simulink model "MPPT_p0x26oPartIALShadingFD"  (R2024b)
settings: Solver=VariableStepAuto  StartTime=0.0  StopTime=1  FixedStep=1e-6  RelTol=1e-4
libraries: spsDiodeLib x5, spsPVArrayLib x4, spsSeriesRLCBranchLib x4, spsVoltageMeasurementLib x3, spsCurrentMeasurementLib x2, spsMosfetLib x1, simulink x1, sps_lib x1
settings Model: Creator=VICTUS  LastModifiedBy=VICTUS
settings SolverCC: ZeroCrossAlgorithm=Adaptive
settings DebuggingCC: MaskedZcDiagnostic=none  IgnoredZcDiagnostic=none

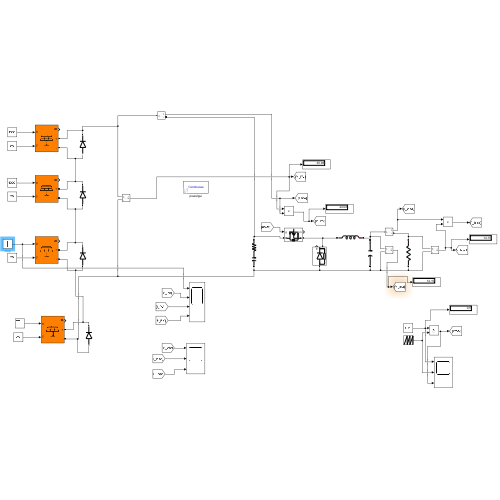
[thumbnail: Simulink's stored preview of the top-level diagram]
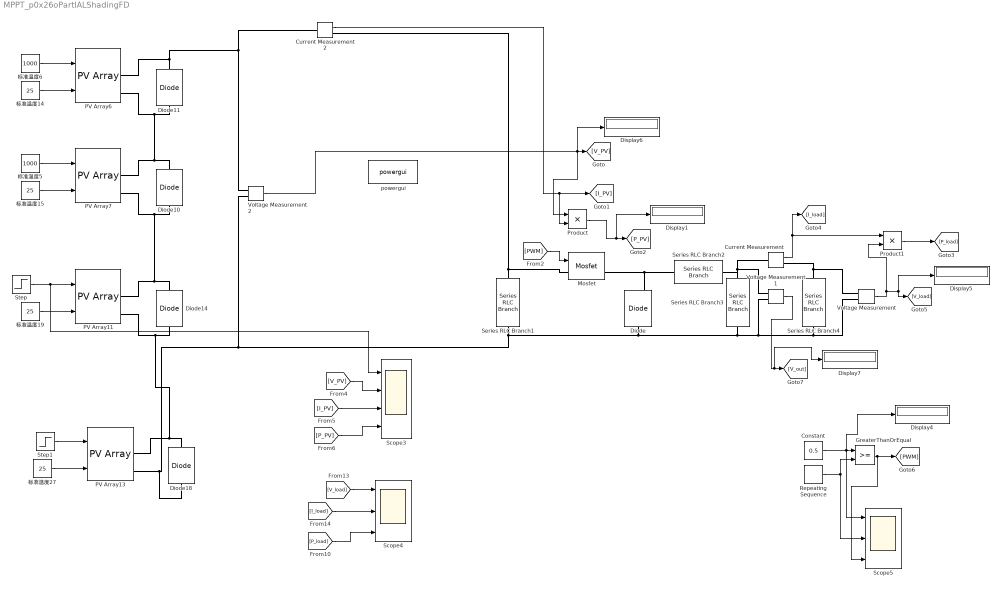
== system MPPT_p0x26oPartIALShadingFD ==
  Constant : Constant  Value=0.5
  Current Measurement : spsCurrentMeasurementLib/Current Measurement  PhasorSimulation=off  OutputType=Complex  PSBequivalent=0
  Current Measurement2 : spsCurrentMeasurementLib/Current Measurement  PhasorSimulation=off  OutputType=Complex  PSBequivalent=0
  Diode : spsDiodeLib/Diode  Ron=0.001  Lon=0  Vf=0.8  IC=0  UseSnubber=0  Rs=500  Cs=250e-9  Measurements=on
  Diode{10..11,14,18} (4 alike) : spsDiodeLib/Diode  Ron=0.001  Lon=0  Vf=0.8  IC=0  UseSnubber=off  Rs=inf  Cs=250e-9  Measurements=off
  Display{1,4..7} (5 alike) : Display
  GreaterThanOrEqual : RelationalOperator  OutDataTypeStr=boolean  RndMeth=Simplest  InputSameDT=off
  Mosfet : spsMosfetLib/Mosfet  Ron=0.1  Lon=0  Rd=0.01  Vfd=0  IC=0  Rs=1e5  Cs=inf  Measurements=on
  PV Array{6..7,11,13} (4 alike) : spsPVArrayLib/PV Array  Npar=1  Nser=1  PlotType=array @ 1000 W/m2 & specified temperatures  S_vec="[ 1000  500  100 ]"  Temp_C_vec="[ 45 25  ]"  ModuleName=User-defined  PlotWhenSelected=off  Pm=120.75  Ncell=16  Voc=22  Isc=7.5  Vm=17.5  Im=6.9  beta_Voc_pc=-0.36099  alpha_Isc_pc=0.102  beta_Voc=-0.079418  alpha_Isc=0.00765  IL=7.6829  I0=2.1898e-10  nI=2.2089  Rsh=50.0358  Rs=0.26399  RobustModel=off  RobustCellTemperature=313.3991  BAL=off  Tc=1e-6  Tfilter=5e-5
  Product : Product
  Product1 : Product
  Repeating Sequence : simulink/Sources/Repeating Sequence  rep_seq_t=[0 2e-4]  rep_seq_y=[0 1]
  Scope3 : Scope  NumInputPorts=4
  Scope4 : Scope  NumInputPorts=3
  Scope5 : Scope  NumInputPorts=3
  Series RLC Branch1 : spsSeriesRLCBranchLib/Series RLC Branch  LConnTagsString=__new0  RConnTagsString=__new0  BranchType=RC  Resistance=0.001  Inductance=1e-3  SetiL0=off  InitialCurrent=0  Capacitance=338e-6  Setx0=off  InitialVoltage=0  Measurements=None
  Series RLC Branch2 : spsSeriesRLCBranchLib/Series RLC Branch  LConnTagsString=__new0  RConnTagsString=__new0  BranchType=L  Resistance=0.001  Inductance=1.25e-3  SetiL0=off  InitialCurrent=0  Capacitance=1000e-6  Setx0=off  InitialVoltage=0  Measurements=None
  Series RLC Branch3 : spsSeriesRLCBranchLib/Series RLC Branch  LConnTagsString=__new0  RConnTagsString=__new0  BranchType=C  Resistance=0.001  Inductance=1e-3  SetiL0=off  InitialCurrent=0  Capacitance=187.5e-6  Setx0=off  InitialVoltage=0  Measurements=None
  Series RLC Branch4 : spsSeriesRLCBranchLib/Series RLC Branch  LConnTagsString=__new0  RConnTagsString=__new0  BranchType=R  Resistance=1  Inductance=1e-3  SetiL0=off  InitialCurrent=0  Capacitance=1000e-6  Setx0=off  InitialVoltage=0  Measurements=None
  Step : Step  Time=0.5  Before=1000  After=400  SampleTime=0
  Step1 : Step  Time=0.5  Before=1000  After=400  SampleTime=0
  Voltage Measurement : spsVoltageMeasurementLib/Voltage Measurement  PhasorSimulation=off  OutputType=Complex  PSBequivalent=0
  Voltage Measurement1 : spsVoltageMeasurementLib/Voltage Measurement  PhasorSimulation=off  OutputType=Complex  PSBequivalent=0
  Voltage Measurement2 : spsVoltageMeasurementLib/Voltage Measurement  PhasorSimulation=off  OutputType=Complex  PSBequivalent=0
  powergui : sps_lib/powergui  Priority=1  SimulationMode=Continuous  SampleTime=50e-6  frequency=60  Iterations=50  frequencyindice=0  Pbase=100e6  ErrMax=1e-4  UnitsV=kV  UnitsW=MW  buscounter=0  FunctionMessages=off  echomessages=off  EnableUseOfTLC=off  CurrentSourceSwitches=off  DisableSnubberDevices=off  DisableRonSwitches=off  DisableVfSwitches=off  DisplayEquations=off  AutomaticDiscreteSolvers=off  SolverType=Tustin/Backward Euler (TBE)  Interpol=off  ExternalGateDelay=off  methode=off  Ts=100  x0status=blocks  SPID=on  SwTol=0  HookPort=off  NonlinearTolerance=1e-4  nMaxIteration=100  ContinueOnMaxIteration=off  RestoreLinks=warning  ResistiveCurrentMeasurement=off  Frange=[0:2:500]  Ylog=off  Xlog=on  ShowGrid=off  save=off  variable=ZData  structure=0  ZoomFFT=off  StartTime=0.0  cycles=1  DisplayStyle=1  fundamental=60  FreqAxis=off  MaxFrequency=1000  frequencyindicesteady=1  RmsSteady=1  display=off
  标准温度{14..15,19,27} (4 alike) : Constant  Value=25  SampleTime=0.001
  标准温度5 : Constant  Value=1000  SampleTime=0.001
  标准温度6 : Constant  Value=1000  SampleTime=0.001
  wires:
  标准温度5/1 -> PV Array7/1
  [V_load] -> Scope4/1
  [PWM] -> Mosfet/1
  Product1/1 -> [P_load]
  [I_PV] -> Scope3/3
  Voltage Measurement2/1 -> Product/1, Display6/1, [V_PV]
  标准温度14/1 -> PV Array6/2
  Voltage Measurement/1 -> Product1/2, Display5/1, [V_load]
  [I_load] -> Scope4/2
  标准温度27/1 -> PV Array13/2
  Current Measurement/1 -> [I_load], Product1/1
  Current Measurement2/1 -> Product/2, [I_PV]
  标准温度15/1 -> PV Array7/2
  标准温度6/1 -> PV Array6/1
  [P_load] -> Scope4/3
  Step/1 -> Scope3/1, PV Array11/1
  Product/1 -> Display1/1, [P_PV]
  标准温度19/1 -> PV Array11/2
  [V_PV] -> Scope3/2
  Voltage Measurement1/1 -> Display7/1, [V_out]
  [P_PV] -> Scope3/4
  Step1/1 -> PV Array13/1
  GreaterThanOrEqual/1 -> Scope5/3, [PWM]
  Repeating Sequence/1 -> Scope5/2, GreaterThanOrEqual/2
  Constant/1 -> Scope5/1, GreaterThanOrEqual/1, Display4/1
  connections:
  Voltage Measurement2/LConn1 -- PV Array6/RConn1 -- Diode11/RConn1 -- Current Measurement2/LConn1
  Voltage Measurement/LConn1 -- Series RLC Branch4/LConn1 -- Current Measurement/RConn1
  PV Array7/RConn2 -- Diode14/RConn1 -- PV Array11/RConn1 -- Diode10/LConn1
  Series RLC Branch2/RConn1 -- Diode/RConn1 -- Mosfet/RConn1
  Series RLC Branch3/LConn1 -- Current Measurement/LConn1 -- Series RLC Branch2/LConn1 -- Voltage Measurement1/LConn1
  Series RLC Branch4/RConn1 -- Series RLC Branch3/RConn1 -- Voltage Measurement2/LConn2 -- PV Array13/RConn2 -- Diode18/LConn1 -- Series RLC Branch1/RConn1 -- Diode/LConn1 -- Voltage Measurement1/LConn2 -- Voltage Measurement/LConn2
  Mosfet/LConn1 -- Series RLC Branch1/LConn1 -- Current Measurement2/RConn1
  PV Array11/RConn2 -- Diode14/LConn1 -- PV Array13/RConn1 -- Diode18/RConn1
  PV Array7/RConn1 -- PV Array6/RConn2 -- Diode11/LConn1 -- Diode10/RConn1
